simulink library "mfeval_CPI_LIB"  (R2026a)
settings: Solver=VariableStepAuto
undefined symbols (not defined in the file or in its folder): parameterStruct, userDynamics, userUseMode
Description:
  | Copyright 2020-2024 The MathWorks, Inc.
settings Model: Creator=MFURLANT  LastModifiedBy=andrei

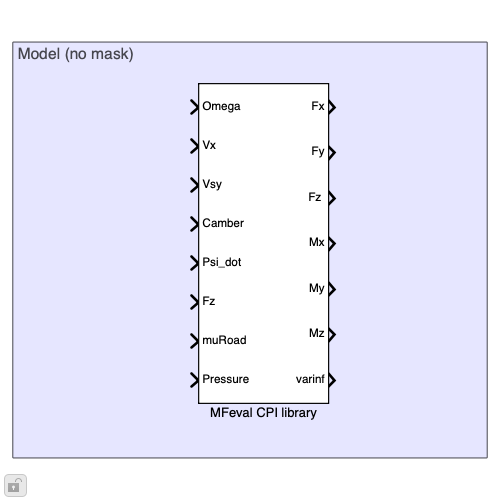
[thumbnail: Simulink's stored preview of the top-level diagram]
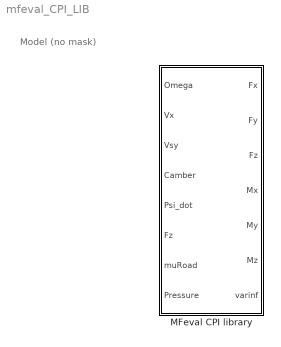
== system mfeval_CPI_LIB ==
  note: Model (no mask)
  MFeval CPI library : Subsystem

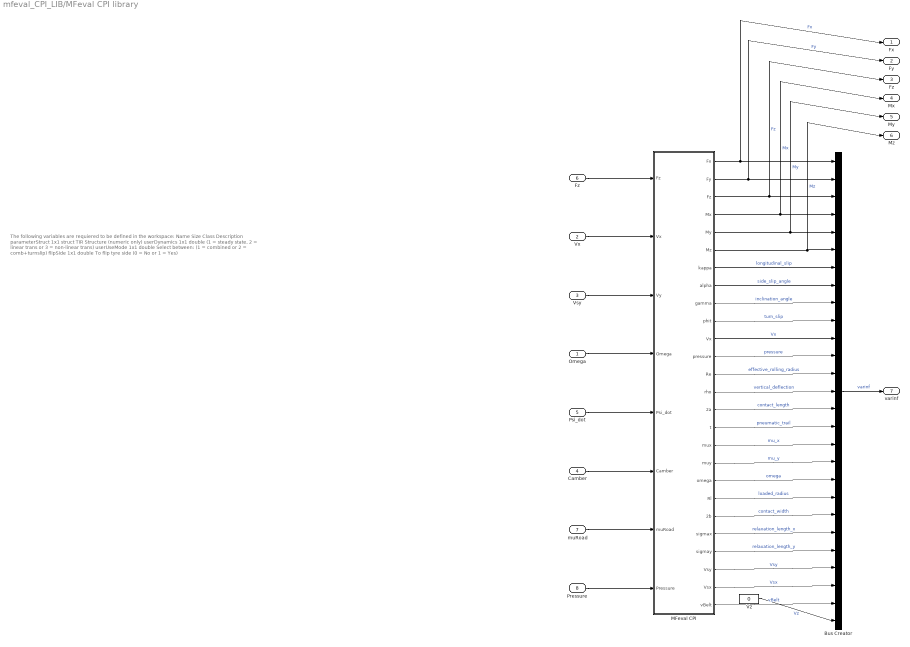
== system mfeval_CPI_LIB/MFeval CPI library ==
  note: The following variables are requiered to be defined in the workspace:
      |
      | Name
      | Size
      | Class
      | Description
      |
      | parameterStruct
      | 1x1
      | struct
      | TIR Structure (numeric only)
      |
      | userDynamics
      | 1x1
      | double
      | (1 = steady state, 2 = linear trans or 3 = non-linear trans)
      |
      | userUseMode
      | 1x1
      | double
      | Select between: (1 = combined or 2 = comb+turnslip)
      |
      | flipSide
      | 1x1
      | double
      | To flip tyre side (0 = No or 1 = Yes)
  Omega : Inport
  Vx : Inport  Port=2
  Vsy : Inport  Port=3
  Camber : Inport  Port=4
  Psi_dot : Inport  Port=5
  Fz : Inport  Port=6
  muRoad : Inport  Port=7
  Pressure : Inport  Port=8
  Bus Creator : BusCreator  Inputs=27
  MFeval CPI : Subsystem
  Vz : Constant  Value=0
  Fx : Outport  VectorParamsAs1DForOutWhenUnconnected=off
  Fy : Outport  Port=2  VectorParamsAs1DForOutWhenUnconnected=off
  "Fz " : Outport  Port=3  VectorParamsAs1DForOutWhenUnconnected=off
  Mx : Outport  Port=4  VectorParamsAs1DForOutWhenUnconnected=off
  My : Outport  Port=5  VectorParamsAs1DForOutWhenUnconnected=off
  Mz : Outport  Port=6  VectorParamsAs1DForOutWhenUnconnected=off
  varinf : Outport  Port=7  VectorParamsAs1DForOutWhenUnconnected=off
  wires:
  Vx/1 -> MFeval CPI/2(Vx)
  MFeval CPI/25(Vsx) -> Bus Creator/25  "Vsx"
  MFeval CPI/13(Re) -> Bus Creator/13  "effective_rolling_radius"
  MFeval CPI/3("Fz ") -> "Fz "/1, Bus Creator/3  "Fz"
  MFeval CPI/22(sigmax) -> Bus Creator/22  "relaxation_length_x"
  MFeval CPI/16(t) -> Bus Creator/16  "pneumatic_trail"
  MFeval CPI/4(Mx) -> Mx/1, Bus Creator/4  "Mx"
  MFeval CPI/6(Mz) -> Mz/1, Bus Creator/6  "Mz"
  MFeval CPI/17(mux) -> Bus Creator/17  "mu_x"
  Vz/1 -> Bus Creator/27  "Vz"
  MFeval CPI/21(2b) -> Bus Creator/21  "contact_width"
  MFeval CPI/1(Fx) -> Fx/1, Bus Creator/1  "Fx"
  MFeval CPI/18(muy) -> Bus Creator/18  "mu_y"
  MFeval CPI/23(sigmay) -> Bus Creator/23  "relaxation_length_y"
  MFeval CPI/8(alpha) -> Bus Creator/8  "side_slip_angle"
  MFeval CPI/7(kappa) -> Bus Creator/7  "longitudinal_slip"
  MFeval CPI/20(Rl) -> Bus Creator/20  "loaded_radius"
  MFeval CPI/15(2a) -> Bus Creator/15  "contact_length"
  MFeval CPI/19(omega) -> Bus Creator/19  "omega"
  MFeval CPI/11("Vx ") -> Bus Creator/11  "Vx"
  MFeval CPI/14(rho) -> Bus Creator/14  "vertical_deflection"
  Fz/1 -> MFeval CPI/1(Fz)
  Bus Creator/1 -> varinf/1  "varinf"
  Camber/1 -> MFeval CPI/6(Camber)
  MFeval CPI/26(vBelt) -> Bus Creator/26  "vBelt"
  MFeval CPI/9(gamma) -> Bus Creator/9  "inclination_angle"
  Omega/1 -> MFeval CPI/4(Omega)
  MFeval CPI/10(phit) -> Bus Creator/10  "turn_slip"
  MFeval CPI/24(Vsy) -> Bus Creator/24  "Vsy"
  MFeval CPI/2(Fy) -> Fy/1, Bus Creator/2  "Fy"
  Psi_dot/1 -> MFeval CPI/5(Psi_dot)
  MFeval CPI/5(My) -> My/1, Bus Creator/5  "My"
  MFeval CPI/12(pressure) -> Bus Creator/12  "pressure"
  Vsy/1 -> MFeval CPI/3(Vy)
  muRoad/1 -> MFeval CPI/7(muRoad)
  Pressure/1 -> MFeval CPI/8(Pressure)

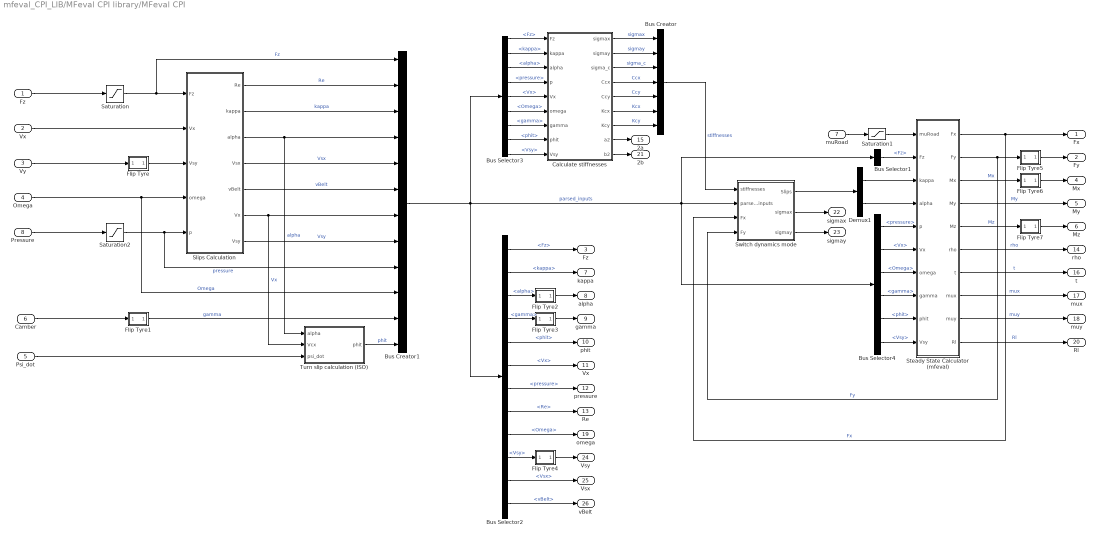
== system mfeval_CPI_LIB/MFeval CPI library/MFeval CPI ==
  Fz : Inport
  Vx : Inport  Port=2
  Vy : Inport  Port=3
  Omega : Inport  Port=4
  Psi_dot : Inport  Port=5
  Camber : Inport  Port=6
  muRoad : Inport  Port=7
  Pressure : Inport  Port=8
  Bus Creator : BusCreator  Inputs=7
  Bus Creator1 : BusCreator  Inputs=12
  Bus Selector1 : BusSelector  OutputSignals=Fz
  Bus Selector2 : BusSelector  OutputSignals=Fz,kappa,alpha,gamma,phit,Vx,pressure,Re,Omega,Vsy,Vsx,vBelt
  Bus Selector3 : BusSelector  OutputSignals=Fz,kappa,alpha,pressure,Vx,Omega,gamma,phit,Vsy
  Bus Selector4 : BusSelector  OutputSignals=pressure,Vx,Omega,gamma,phit,Vsy
  Calculate stiffnesses : MATLAB Function  TreatAsAtomicUnit=on
  Demux1 : Demux  Outputs=2
  Flip Tyre : MATLAB Function  TreatAsAtomicUnit=on
  Flip Tyre1 : MATLAB Function  TreatAsAtomicUnit=on
  Flip Tyre2 : MATLAB Function  TreatAsAtomicUnit=on
  Flip Tyre3 : MATLAB Function  TreatAsAtomicUnit=on
  Flip Tyre4 : MATLAB Function  TreatAsAtomicUnit=on
  Flip Tyre5 : MATLAB Function  TreatAsAtomicUnit=on
  Flip Tyre6 : MATLAB Function  TreatAsAtomicUnit=on
  Flip Tyre7 : MATLAB Function  TreatAsAtomicUnit=on
  Saturation : Saturate  UpperLimit=parameterStruct.FZMAX*2  LowerLimit=1e-3  ZeroCross=off
  Saturation1 : Saturate  UpperLimit=Inf  LowerLimit=0  ZeroCross=off
  Saturation2 : Saturate  UpperLimit=parameterStruct.PRESMAX  LowerLimit=parameterStruct.PRESMIN  ZeroCross=off
  Slips Calculation : MATLAB Function  TreatAsAtomicUnit=on
  Steady State Calculator (mfeval) : MATLAB Function  TreatAsAtomicUnit=on
  Switch dynamics mode : Subsystem
  Turn slip calculation (ISO) : MATLAB Function  TreatAsAtomicUnit=on
  Fx : Outport  VectorParamsAs1DForOutWhenUnconnected=off
  Fy : Outport  Port=2  VectorParamsAs1DForOutWhenUnconnected=off
  "Fz " : Outport  Port=3  VectorParamsAs1DForOutWhenUnconnected=off
  Mx : Outport  Port=4  VectorParamsAs1DForOutWhenUnconnected=off
  My : Outport  Port=5  VectorParamsAs1DForOutWhenUnconnected=off
  Mz : Outport  Port=6  VectorParamsAs1DForOutWhenUnconnected=off
  kappa : Outport  Port=7  VectorParamsAs1DForOutWhenUnconnected=off
  alpha : Outport  Port=8  VectorParamsAs1DForOutWhenUnconnected=off
  gamma : Outport  Port=9  VectorParamsAs1DForOutWhenUnconnected=off
  phit : Outport  Port=10  VectorParamsAs1DForOutWhenUnconnected=off
  "Vx " : Outport  Port=11  VectorParamsAs1DForOutWhenUnconnected=off
  pressure : Outport  Port=12  VectorParamsAs1DForOutWhenUnconnected=off
  Re : Outport  Port=13  VectorParamsAs1DForOutWhenUnconnected=off
  rho : Outport  Port=14  VectorParamsAs1DForOutWhenUnconnected=off
  2a : Outport  Port=15  VectorParamsAs1DForOutWhenUnconnected=off
  t : Outport  Port=16  VectorParamsAs1DForOutWhenUnconnected=off
  mux : Outport  Port=17  VectorParamsAs1DForOutWhenUnconnected=off
  muy : Outport  Port=18  VectorParamsAs1DForOutWhenUnconnected=off
  omega : Outport  Port=19  VectorParamsAs1DForOutWhenUnconnected=off
  Rl : Outport  Port=20  VectorParamsAs1DForOutWhenUnconnected=off
  2b : Outport  Port=21  VectorParamsAs1DForOutWhenUnconnected=off
  sigmax : Outport  Port=22  VectorParamsAs1DForOutWhenUnconnected=off
  sigmay : Outport  Port=23  VectorParamsAs1DForOutWhenUnconnected=off
  Vsy : Outport  Port=24  VectorParamsAs1DForOutWhenUnconnected=off
  Vsx : Outport  Port=25  VectorParamsAs1DForOutWhenUnconnected=off
  vBelt : Outport  Port=26  VectorParamsAs1DForOutWhenUnconnected=off
  wires:
  Pressure/1 -> Saturation2/1
  Camber/1 -> Flip Tyre1/1(in)
  Turn slip calculation (ISO)/1(phit) -> Bus Creator1/12  "phit"
  Vx/1 -> Slips Calculation/2("Vx ")
  Steady State Calculator (mfeval)/9(muy) -> muy/1  "muy"
  Steady State Calculator (mfeval)/5(Mz) -> Flip Tyre7/1(in)  "Mz"
  Vy/1 -> Flip Tyre/1(in)
  Steady State Calculator (mfeval)/3(Mx) -> Flip Tyre6/1(in)  "Mx"
  Slips Calculation/2(kappa) -> Bus Creator1/3  "kappa"
  Steady State Calculator (mfeval)/7(t) -> t/1  "t"
  Steady State Calculator (mfeval)/4(My) -> My/1  "My"
  Steady State Calculator (mfeval)/8(mux) -> mux/1  "mux"
  Steady State Calculator (mfeval)/6(rho) -> rho/1  "rho"
  Fz/1 -> Saturation/1
  Omega/1 -> Bus Creator1/10, Slips Calculation/4(omega)  "Omega"
  Psi_dot/1 -> Turn slip calculation (ISO)/3(psi_dot)
  Slips Calculation/4(Vsx) -> Bus Creator1/5  "Vsx"
  Bus Selector3/1 -> Calculate stiffnesses/1(Fz)  "<Fz>"
  Bus Selector3/2 -> Calculate stiffnesses/2(kappa)  "<kappa>"
  Bus Selector3/3 -> Calculate stiffnesses/3(alpha)  "<alpha>"
  Bus Selector3/4 -> Calculate stiffnesses/4(p)  "<pressure>"
  Bus Selector3/5 -> Calculate stiffnesses/5(Vx)  "<Vx>"
  Bus Selector3/6 -> Calculate stiffnesses/6(omega)  "<Omega>"
  Bus Selector3/7 -> Calculate stiffnesses/7(gamma)  "<gamma>"
  Bus Selector3/8 -> Calculate stiffnesses/8(phit)  "<phit>"
  Calculate stiffnesses/1(sigmax) -> Bus Creator/1  "sigmax"
  Calculate stiffnesses/2(sigmay) -> Bus Creator/2  "sigmay"
  Calculate stiffnesses/3(sigma_c) -> Bus Creator/3  "sigma_c"
  Calculate stiffnesses/4(Ccx) -> Bus Creator/4  "Ccx"
  Calculate stiffnesses/5(Ccy) -> Bus Creator/5  "Ccy"
  Calculate stiffnesses/6(Kcx) -> Bus Creator/6  "Kcx"
  Calculate stiffnesses/7(Kcy) -> Bus Creator/7  "Kcy"
  Bus Creator1/1 -> Bus Selector3/1, Bus Selector1/1, Switch dynamics mode/2(parsed_inputs), Bus Selector4/1, Bus Selector2/1  "parsed_inputs"
  Demux1/2 -> Steady State Calculator (mfeval)/4(alpha)
  Slips Calculation/3(alpha) -> Turn slip calculation (ISO)/1(alpha), Bus Creator1/4  "alpha"
  Flip Tyre2/1(out) -> alpha/1
  Flip Tyre1/1(out) -> Bus Creator1/11  "gamma"
  Flip Tyre3/1(out) -> gamma/1
  Flip Tyre6/1(out) -> Mx/1
  Flip Tyre7/1(out) -> Mz/1
  Flip Tyre5/1(out) -> Fy/1
  Flip Tyre/1(out) -> Slips Calculation/3("Vsy ")
  Flip Tyre4/1(out) -> Vsy/1
  Steady State Calculator (mfeval)/2(Fy) -> Switch dynamics mode/4(Fy), Flip Tyre5/1(in)  "Fy"
  Steady State Calculator (mfeval)/1(Fx) -> Switch dynamics mode/3(Fx), Fx/1  "Fx"
  Switch dynamics mode/1(Slips) -> Demux1/1
  Slips Calculation/6(Vx) -> Turn slip calculation (ISO)/2(Vcx), Bus Creator1/7  "Vx"
  Slips Calculation/7(Vsy) -> Bus Creator1/8  "Vsy"
  Calculate stiffnesses/8(a2) -> 2a/1
  Slips Calculation/1(Re) -> Bus Creator1/2  "Re"
  Slips Calculation/5(vBelt) -> Bus Creator1/6  "vBelt"
  Bus Selector2/1 -> "Fz "/1  "<Fz>"
  Bus Selector2/12 -> vBelt/1  "<vBelt>"
  Bus Selector2/2 -> kappa/1  "<kappa>"
  Bus Selector2/3 -> Flip Tyre2/1(in)  "<alpha>"
  Bus Selector2/4 -> Flip Tyre3/1(in)  "<gamma>"
  Bus Selector2/5 -> phit/1  "<phit>"
  Bus Selector2/6 -> "Vx "/1  "<Vx>"
  Bus Selector2/7 -> pressure/1  "<pressure>"
  Bus Selector2/8 -> Re/1  "<Re>"
  Bus Selector2/9 -> omega/1  "<Omega>"
  Bus Selector2/10 -> Flip Tyre4/1(in)  "<Vsy>"
  Bus Selector2/11 -> Vsx/1  "<Vsx>"
  Steady State Calculator (mfeval)/10(Rl) -> Rl/1  "Rl"
  Calculate stiffnesses/9(b2) -> 2b/1
  Bus Selector3/9 -> Calculate stiffnesses/9(Vsy)  "<Vsy>"
  Demux1/1 -> Steady State Calculator (mfeval)/3(kappa)
  Saturation/1 -> Bus Creator1/1, Slips Calculation/1(Fz)  "Fz"
  Bus Creator/1 -> Switch dynamics mode/1(stiffnesses)  "stiffnesses"
  Switch dynamics mode/2(sigmax) -> sigmax/1
  Switch dynamics mode/3(sigmay) -> sigmay/1
  Bus Selector1/1 -> Steady State Calculator (mfeval)/2(Fz)  "<Fz>"
  Bus Selector4/1 -> Steady State Calculator (mfeval)/5(p)  "<pressure>"
  Bus Selector4/2 -> Steady State Calculator (mfeval)/6(Vx)  "<Vx>"
  Bus Selector4/3 -> Steady State Calculator (mfeval)/7(omega)  "<Omega>"
  Bus Selector4/4 -> Steady State Calculator (mfeval)/8(gamma)  "<gamma>"
  Bus Selector4/5 -> Steady State Calculator (mfeval)/9(phit)  "<phit>"
  Bus Selector4/6 -> Steady State Calculator (mfeval)/10(Vsy)  "<Vsy>"
  muRoad/1 -> Saturation1/1
  Saturation1/1 -> Steady State Calculator (mfeval)/1(muRoad)
  Saturation2/1 -> Bus Creator1/9, Slips Calculation/5(p)  "pressure"

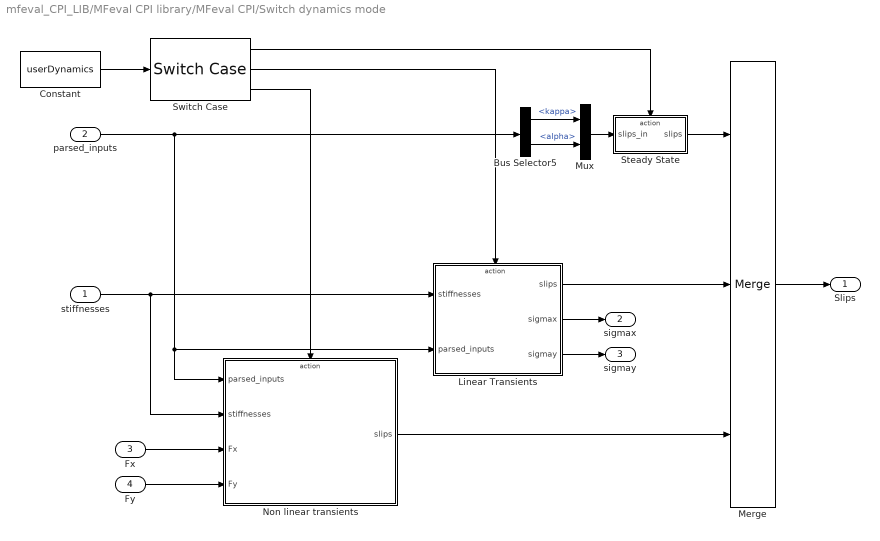
== system mfeval_CPI_LIB/MFeval CPI library/MFeval CPI/Switch dynamics mode ==
  stiffnesses : Inport
  parsed_inputs : Inport  Port=2
  Fx : Inport  Port=3
  Fy : Inport  Port=4
  Bus Selector5 : BusSelector  OutputSignals=kappa,alpha
  Constant : Constant  Value=userDynamics
  Linear Transients : Subsystem  TreatAsAtomicUnit=on
  Merge : Merge  Inputs=3
  Mux : Mux  Inputs=2
  Non linear transients : Subsystem  TreatAsAtomicUnit=on
  Steady State : Subsystem  TreatAsAtomicUnit=on
  Switch Case : SwitchCase  CaseConditions={1, 2}
  Slips : Outport  VectorParamsAs1DForOutWhenUnconnected=off
  sigmax : Outport  Port=2  VectorParamsAs1DForOutWhenUnconnected=off
  sigmay : Outport  Port=3  VectorParamsAs1DForOutWhenUnconnected=off
  wires:
  Constant/1 -> Switch Case/1
  Switch Case/1 -> Steady State/Action
  Switch Case/2 -> Linear Transients/Action
  Linear Transients/1(slips) -> Merge/2
  Switch Case/3 -> Non linear transients/Action
  Non linear transients/1(slips) -> Merge/3
  Steady State/1(slips) -> Merge/1
  Merge/1 -> Slips/1
  parsed_inputs/1 -> Bus Selector5/1, Non linear transients/1(parsed_inputs), Linear Transients/2(parsed_inputs)
  Fx/1 -> Non linear transients/3(Fx)
  Fy/1 -> Non linear transients/4(Fy)
  stiffnesses/1 -> Non linear transients/2(stiffnesses), Linear Transients/1(stiffnesses)
  Linear Transients/2(sigmax) -> sigmax/1
  Linear Transients/3(sigmay) -> sigmay/1
  Bus Selector5/2 -> Mux/2  "<alpha>"
  Bus Selector5/1 -> Mux/1  "<kappa>"
  Mux/1 -> Steady State/1(slips_in)

== system mfeval_CPI_LIB/MFeval CPI library/MFeval CPI/Switch dynamics mode/Linear Transients ==
  stiffnesses : Inport
  parsed_inputs : Inport  Port=2
  Action Port : ActionPort  ActionPortLabel=case: { }
  Bus Selector : BusSelector  OutputSignals=sigmax,sigmay
  Bus Selector5 : BusSelector  OutputSignals=Vsx,Vsy,Vx
  Calculate Slips : Subsystem  TreatAsAtomicUnit=on
  Mux1 : Mux  Inputs=2
  slips : Outport  VectorParamsAs1DForOutWhenUnconnected=off
  sigmax : Outport  Port=2  VectorParamsAs1DForOutWhenUnconnected=off
  sigmay : Outport  Port=3  VectorParamsAs1DForOutWhenUnconnected=off
  wires:
  Calculate Slips/2(alpha) -> Mux1/2
  Mux1/1 -> slips/1  "Linear transients"
  Bus Selector/2 -> sigmay/1, Calculate Slips/2(sigmay)  "<sigmay>"
  Bus Selector5/3 -> Calculate Slips/5(Vx)  "<Vx>"
  Calculate Slips/1(kappa) -> Mux1/1
  Bus Selector5/2 -> Calculate Slips/4(Vsy)  "<Vsy>"
  Bus Selector5/1 -> Calculate Slips/3(Vsx)  "<Vsx>"
  Bus Selector/1 -> sigmax/1, Calculate Slips/1(sigmax)  "<sigmax>"
  stiffnesses/1 -> Bus Selector/1  "stiffnesses"
  parsed_inputs/1 -> Bus Selector5/1

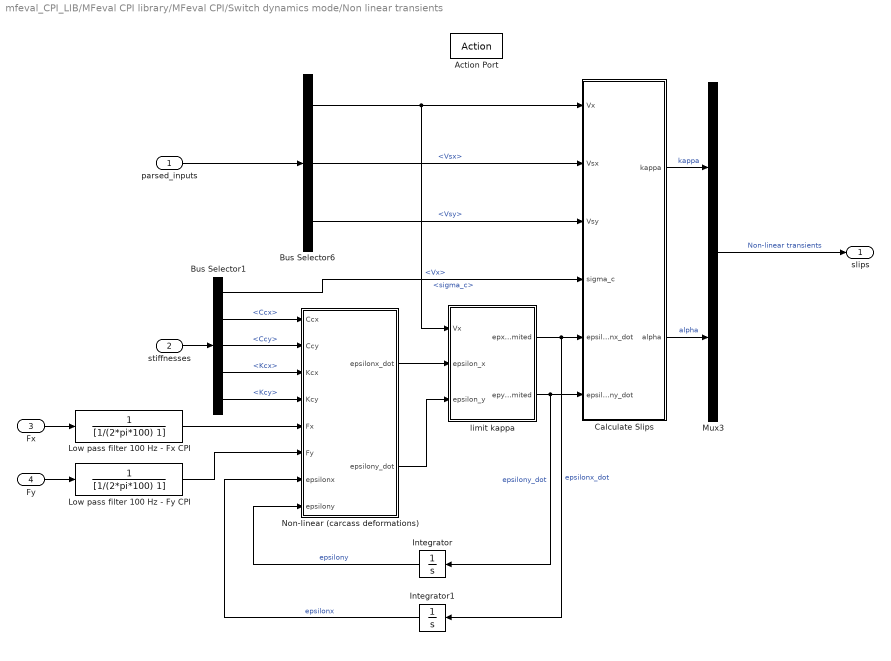
== system mfeval_CPI_LIB/MFeval CPI library/MFeval CPI/Switch dynamics mode/Non linear transients ==
  parsed_inputs : Inport
  stiffnesses : Inport  Port=2
  Fx : Inport  Port=3
  Fy : Inport  Port=4
  Action Port : ActionPort  ActionPortLabel=default: { }
  Bus Selector1 : BusSelector  OutputSignals=sigma_c,Ccx,Ccy,Kcx,Kcy
  Bus Selector6 : BusSelector  OutputSignals=Vx,Vsx,Vsy
  Calculate Slips : Subsystem  TreatAsAtomicUnit=on
  Integrator : Integrator
  Integrator1 : Integrator
  Low pass filter 100 Hz - Fx CPI : TransferFcn  Denominator=[1/(2*pi*100) 1]
  Low pass filter 100 Hz - Fy CPI : TransferFcn  Denominator=[1/(2*pi*100) 1]
  Mux3 : Mux  Inputs=2
  Non-linear (carcass deformations) : Subsystem
  limit kappa : Subsystem
  slips : Outport  VectorParamsAs1DForOutWhenUnconnected=off
  wires:
  Calculate Slips/1(kappa) -> Mux3/1  "kappa"
  Mux3/1 -> slips/1  "Non-linear transients"
  Non-linear (carcass deformations)/1(epsilonx_dot) -> limit kappa/2(epsilon_x)
  Bus Selector1/5 -> Non-linear (carcass deformations)/4(Kcy)  "<Kcy>"
  Bus Selector6/2 -> Calculate Slips/2(Vsx)  "<Vsx>"
  Integrator/1 -> Non-linear (carcass deformations)/8(epsilony)  "epsilony"
  Bus Selector1/4 -> Non-linear (carcass deformations)/3(Kcx)  "<Kcx>"
  Calculate Slips/2(alpha) -> Mux3/2  "alpha"
  Non-linear (carcass deformations)/2(epsilony_dot) -> limit kappa/3(epsilon_y)
  Bus Selector6/1 -> limit kappa/1(Vx), Calculate Slips/1(Vx)  "<Vx>"
  limit kappa/2(epy_limited) -> Integrator/1, Calculate Slips/6(epsilony_dot)  "epsilony_dot"
  Bus Selector6/3 -> Calculate Slips/3(Vsy)  "<Vsy>"
  Bus Selector1/2 -> Non-linear (carcass deformations)/1(Ccx)  "<Ccx>"
  Integrator1/1 -> Non-linear (carcass deformations)/7(epsilonx)  "epsilonx"
  Bus Selector1/3 -> Non-linear (carcass deformations)/2(Ccy)  "<Ccy>"
  Bus Selector1/1 -> Calculate Slips/4(sigma_c)  "<sigma_c>"
  limit kappa/1(epx_limited) -> Integrator1/1, Calculate Slips/5(epsilonx_dot)  "epsilonx_dot"
  parsed_inputs/1 -> Bus Selector6/1
  stiffnesses/1 -> Bus Selector1/1
  Fx/1 -> Low pass filter 100 Hz - Fx CPI/1
  Fy/1 -> Low pass filter 100 Hz - Fy CPI/1
  Low pass filter 100 Hz - Fy CPI/1 -> Non-linear (carcass deformations)/6(Fy)
  Low pass filter 100 Hz - Fx CPI/1 -> Non-linear (carcass deformations)/5(Fx)

== system mfeval_CPI_LIB/MFeval CPI library/MFeval CPI/Switch dynamics mode/Steady State ==
  slips_in : Inport
  Action Port : ActionPort  ActionPortLabel=case: { }
  slips : Outport  VectorParamsAs1DForOutWhenUnconnected=off
  wires:
  slips_in/1 -> slips/1

== system mfeval_CPI_LIB/MFeval CPI library/MFeval CPI/Switch dynamics mode/Linear Transients/Calculate Slips ==
  sigmax : Inport
  sigmay : Inport  Port=2
  Vsx : Inport  Port=3
  Vsy : Inport  Port=4
  Vx : Inport  Port=5
  Integrator : Integrator
  Integrator1 : Integrator
  calculate alpha_dot : Subsystem
  calculate kappa_dot : Subsystem
  kappa : Outport  VectorParamsAs1DForOutWhenUnconnected=off
  alpha : Outport  Port=2  VectorParamsAs1DForOutWhenUnconnected=off
  wires:
  Vx/1 -> calculate kappa_dot/1(Vx), calculate alpha_dot/1(Vx)
  Integrator1/1 -> kappa/1, calculate kappa_dot/4(kappa)  "kappa"
  Integrator/1 -> alpha/1, calculate alpha_dot/4(alpha)  "alpha"
  calculate kappa_dot/1(kappa_dot) -> Integrator1/1  "kappa_dot"
  calculate alpha_dot/1(alpha_dot) -> Integrator/1  "alpha_dot"
  sigmax/1 -> calculate kappa_dot/3(sigmax)
  Vsy/1 -> calculate alpha_dot/2(Vsy)
  sigmay/1 -> calculate alpha_dot/3(sigmay)
  Vsx/1 -> calculate kappa_dot/2(Vsx)

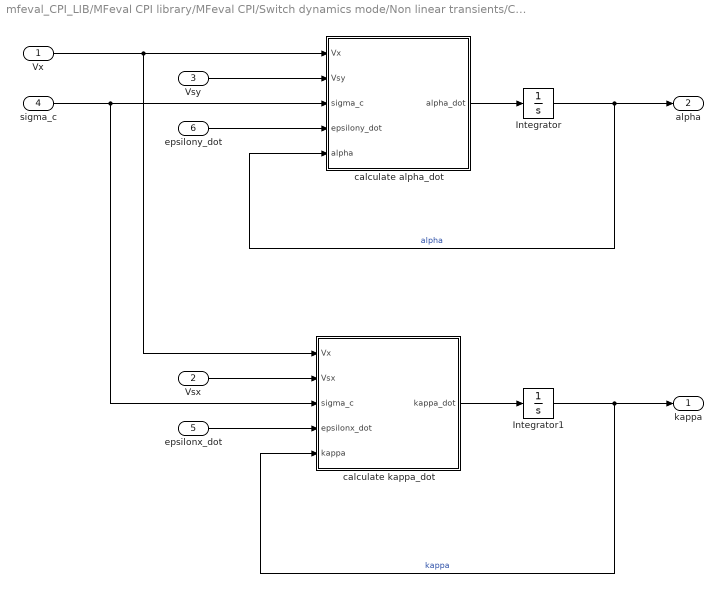
== system mfeval_CPI_LIB/MFeval CPI library/MFeval CPI/Switch dynamics mode/Non linear transients/Calculate Slips ==
  Vx : Inport
  Vsx : Inport  Port=2
  Vsy : Inport  Port=3
  sigma_c : Inport  Port=4
  epsilonx_dot : Inport  Port=5
  epsilony_dot : Inport  Port=6
  Integrator : Integrator
  Integrator1 : Integrator
  calculate alpha_dot : Subsystem
  calculate kappa_dot : Subsystem
  kappa : Outport  VectorParamsAs1DForOutWhenUnconnected=off
  alpha : Outport  Port=2  VectorParamsAs1DForOutWhenUnconnected=off
  wires:
  Integrator1/1 -> calculate kappa_dot/5(kappa), kappa/1  "kappa"
  Integrator/1 -> calculate alpha_dot/5(alpha), alpha/1  "alpha"
  epsilony_dot/1 -> calculate alpha_dot/4(epsilony_dot)
  calculate alpha_dot/1(alpha_dot) -> Integrator/1
  calculate kappa_dot/1(kappa_dot) -> Integrator1/1
  sigma_c/1 -> calculate kappa_dot/3(sigma_c), calculate alpha_dot/3(sigma_c)
  Vsy/1 -> calculate alpha_dot/2(Vsy)
  Vsx/1 -> calculate kappa_dot/2(Vsx)
  epsilonx_dot/1 -> calculate kappa_dot/4(epsilonx_dot)
  Vx/1 -> calculate kappa_dot/1(Vx), calculate alpha_dot/1(Vx)

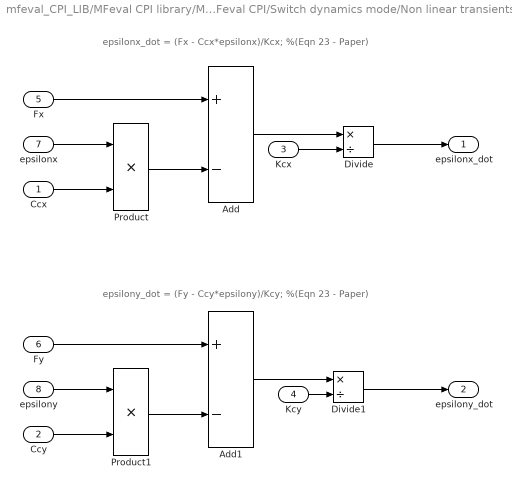
== system mfeval_CPI_LIB/MFeval CPI library/MFeval CPI/Switch dynamics mode/Non linear transients/Non-linear (carcass deformations) ==
  note: epsilony_dot = (Fy - Ccy*epsilony)/Kcy; %(Eqn 23 - Paper)
  note: epsilonx_dot = (Fx - Ccx*epsilonx)/Kcx; %(Eqn 23 - Paper)
  Ccx : Inport
  Ccy : Inport  Port=2
  Kcx : Inport  Port=3
  Kcy : Inport  Port=4
  Fx : Inport  Port=5
  Fy : Inport  Port=6
  epsilonx : Inport  Port=7
  epsilony : Inport  Port=8
  Add : Sum  Inputs=+-
  Add1 : Sum  Inputs=+-
  Divide : Product  Inputs=*/
  Divide1 : Product  Inputs=*/
  Product : Product
  Product1 : Product
  epsilonx_dot : Outport  VectorParamsAs1DForOutWhenUnconnected=off
  epsilony_dot : Outport  Port=2  VectorParamsAs1DForOutWhenUnconnected=off
  wires:
  Fx/1 -> Add/1
  epsilonx/1 -> Product/1
  Ccx/1 -> Product/2
  Product/1 -> Add/2
  Add/1 -> Divide/1
  Kcx/1 -> Divide/2
  Divide/1 -> epsilonx_dot/1
  Ccy/1 -> Product1/2
  epsilony/1 -> Product1/1
  Product1/1 -> Add1/2
  Fy/1 -> Add1/1
  Add1/1 -> Divide1/1
  Kcy/1 -> Divide1/2
  Divide1/1 -> epsilony_dot/1

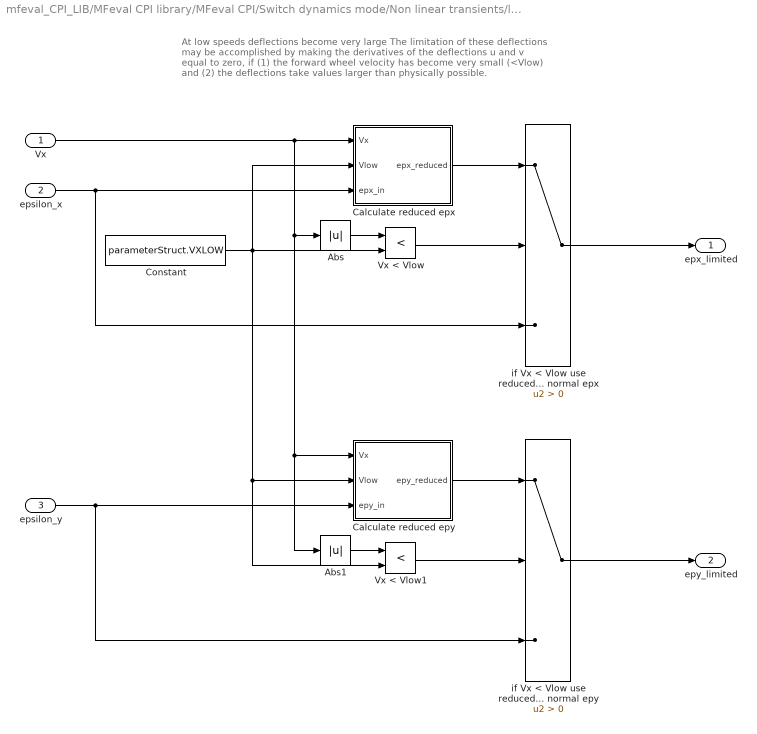
== system mfeval_CPI_LIB/MFeval CPI library/MFeval CPI/Switch dynamics mode/Non linear transients/limit kappa ==
  note: At low speeds deflections become very large
      | The limitation of these deflections may be accomplished by making the
      | derivatives of the deflections u and v equal to zero, if (1) the forward
      | wheel velocity has become very small (<Vlow) and (2) the deflections take
      | values larger than physically possible.
  Vx : Inport
  epsilon_x : Inport  Port=2
  epsilon_y : Inport  Port=3
  Abs : Abs  ZeroCross=off  SaturateOnIntegerOverflow=off
  Abs1 : Abs  ZeroCross=off  SaturateOnIntegerOverflow=off
  Calculate reduced epx : Subsystem
  Calculate reduced epy : Subsystem
  Constant : Constant  Value=parameterStruct.VXLOW
  Vx < Vlow : RelationalOperator  Operator=<  OutDataTypeStr=boolean  ZeroCross=off  RndMeth=Simplest  InputSameDT=off
  Vx < Vlow1 : RelationalOperator  Operator=<  OutDataTypeStr=boolean  ZeroCross=off  RndMeth=Simplest  InputSameDT=off
  if Vx < Vlow use reduced epx else normal epx : Switch  Criteria=u2 > Threshold  SaturateOnIntegerOverflow=off  InputSameDT=off
  if Vx < Vlow use reduced epy else normal epy : Switch  Criteria=u2 > Threshold  SaturateOnIntegerOverflow=off  InputSameDT=off
  epx_limited : Outport  VectorParamsAs1DForOutWhenUnconnected=off
  epy_limited : Outport  Port=2  VectorParamsAs1DForOutWhenUnconnected=off
  wires:
  epsilon_x/1 -> Calculate reduced epx/3(epx_in), if Vx < Vlow use reduced epx else normal epx/3
  if Vx < Vlow use reduced epx else normal epx/1 -> epx_limited/1
  Vx/1 -> Calculate reduced epx/1(Vx), Abs1/1, Calculate reduced epy/1(Vx), Abs/1
  Calculate reduced epx/1(epx_reduced) -> if Vx < Vlow use reduced epx else normal epx/1
  Vx < Vlow/1 -> if Vx < Vlow use reduced epx else normal epx/2
  Calculate reduced epy/1(epy_reduced) -> if Vx < Vlow use reduced epy else normal epy/1
  epsilon_y/1 -> Calculate reduced epy/3(epy_in), if Vx < Vlow use reduced epy else normal epy/3
  Constant/1 -> Vx < Vlow1/2, Calculate reduced epy/2(Vlow), Calculate reduced epx/2(Vlow), Vx < Vlow/2
  if Vx < Vlow use reduced epy else normal epy/1 -> epy_limited/1
  Vx < Vlow1/1 -> if Vx < Vlow use reduced epy else normal epy/2
  Abs/1 -> Vx < Vlow/1
  Abs1/1 -> Vx < Vlow1/1

== system mfeval_CPI_LIB/MFeval CPI library/MFeval CPI/Switch dynamics mode/Linear Transients/Calculate Slips/calculate alpha_dot ==
  note: alpha_dot = (-abs(Vx).*alpha + Vsy)./ max(sigmay, 0.02); % (Eqn 21 - Paper)
  Vx : Inport
  Vsy : Inport  Port=2
  sigmay : Inport  Port=3
  alpha : Inport  Port=4
  Abs : Abs  ZeroCross=off  SaturateOnIntegerOverflow=off
  Add : Sum
  Constant : Constant  Value=0.02
  Divide : Product  Inputs=*/
  Gain : Gain  Gain=-1
  MinMax : MinMax  Function=max  Inputs=2  ZeroCross=off
  Product : Product
  alpha_dot : Outport  VectorParamsAs1DForOutWhenUnconnected=off
  wires:
  Vx/1 -> Abs/1
  alpha/1 -> Product/2
  Abs/1 -> Gain/1
  Product/1 -> Add/1
  Vsy/1 -> Add/2
  Add/1 -> Divide/1
  sigmay/1 -> MinMax/2
  MinMax/1 -> Divide/2
  Constant/1 -> MinMax/1
  Divide/1 -> alpha_dot/1
  Gain/1 -> Product/1

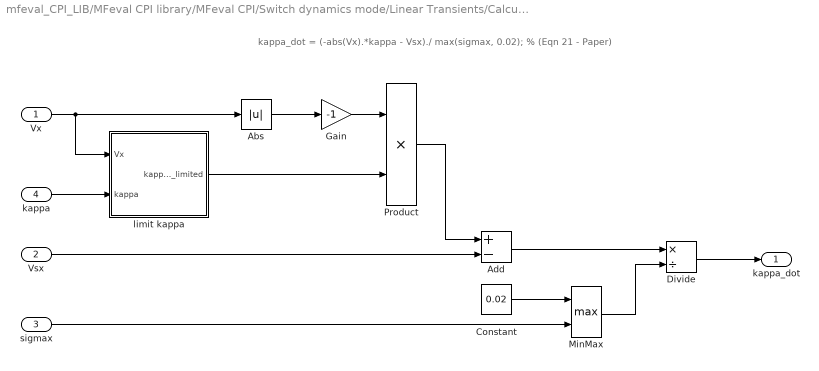
== system mfeval_CPI_LIB/MFeval CPI library/MFeval CPI/Switch dynamics mode/Linear Transients/Calculate Slips/calculate kappa_dot ==
  note: kappa_dot = (-abs(Vx).*kappa - Vsx)./ max(sigmax, 0.02); % (Eqn 21 - Paper)
  Vx : Inport
  Vsx : Inport  Port=2
  sigmax : Inport  Port=3
  kappa : Inport  Port=4
  Abs : Abs  ZeroCross=off  SaturateOnIntegerOverflow=off
  Add : Sum  Inputs=+-
  Constant : Constant  Value=0.02
  Divide : Product  Inputs=*/
  Gain : Gain  Gain=-1
  MinMax : MinMax  Function=max  Inputs=2  ZeroCross=off
  Product : Product
  limit kappa : Subsystem
  kappa_dot : Outport  VectorParamsAs1DForOutWhenUnconnected=off
  wires:
  MinMax/1 -> Divide/2
  Gain/1 -> Product/1
  Constant/1 -> MinMax/1
  Product/1 -> Add/1
  Divide/1 -> kappa_dot/1
  Vsx/1 -> Add/2
  sigmax/1 -> MinMax/2
  Add/1 -> Divide/1
  Abs/1 -> Gain/1
  kappa/1 -> limit kappa/2(kappa)
  Vx/1 -> limit kappa/1(Vx), Abs/1
  limit kappa/1(kappa_limited) -> Product/2

== system mfeval_CPI_LIB/MFeval CPI library/MFeval CPI/Switch dynamics mode/Non linear transients/Calculate Slips/calculate alpha_dot ==
  note: alpha_dot = (-abs(Vx)*alpha + Vsy + epsilony_dot)/ sigma_c; % (Eqn 21 - Paper)
  Vx : Inport
  Vsy : Inport  Port=2
  sigma_c : Inport  Port=3
  epsilony_dot : Inport  Port=4
  alpha : Inport  Port=5
  Abs : Abs  ZeroCross=off  SaturateOnIntegerOverflow=off
  Add : Sum  Inputs=+++
  Divide : Product  Inputs=*/
  Gain : Gain  Gain=-1
  Product : Product
  alpha_dot : Outport  VectorParamsAs1DForOutWhenUnconnected=off
  wires:
  Vx/1 -> Abs/1
  Gain/1 -> Product/1
  Abs/1 -> Gain/1
  alpha/1 -> Product/2
  Product/1 -> Add/1
  Vsy/1 -> Add/2
  epsilony_dot/1 -> Add/3
  Add/1 -> Divide/1
  sigma_c/1 -> Divide/2
  Divide/1 -> alpha_dot/1

== system mfeval_CPI_LIB/MFeval CPI library/MFeval CPI/Switch dynamics mode/Non linear transients/Calculate Slips/calculate kappa_dot ==
  note: kappa_dot = (-abs(Vx).*kappa - (Vsx + epsilonx_dot))./ sigma_c; % (Eqn 21 - Paper)
  Vx : Inport
  Vsx : Inport  Port=2
  sigma_c : Inport  Port=3
  epsilonx_dot : Inport  Port=4
  kappa : Inport  Port=5
  Abs : Abs  ZeroCross=off  SaturateOnIntegerOverflow=off
  Add : Sum
  Add1 : Sum  Inputs=+-
  Divide : Product  Inputs=*/
  Gain : Gain  Gain=-1
  Product : Product
  kappa_dot : Outport  VectorParamsAs1DForOutWhenUnconnected=off
  wires:
  Divide/1 -> kappa_dot/1
  sigma_c/1 -> Divide/2
  Add1/1 -> Divide/1
  epsilonx_dot/1 -> Add/2
  Vsx/1 -> Add/1
  Product/1 -> Add1/1
  kappa/1 -> Product/2
  Abs/1 -> Gain/1
  Gain/1 -> Product/1
  Vx/1 -> Abs/1
  Add/1 -> Add1/2

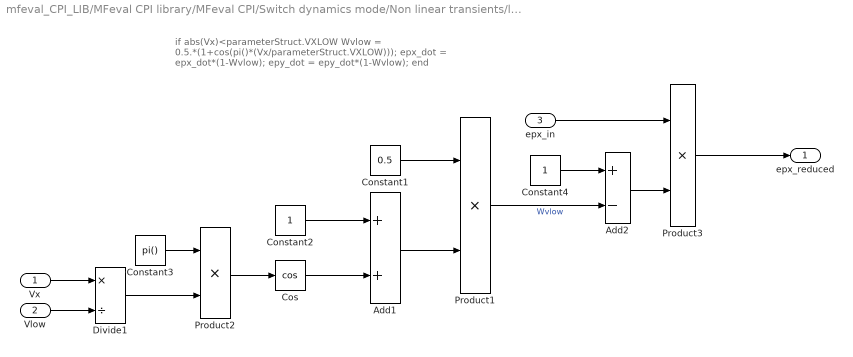
== system mfeval_CPI_LIB/MFeval CPI library/MFeval CPI/Switch dynamics mode/Non linear transients/limit kappa/Calculate reduced epx ==
  note: if abs(Vx)<parameterStruct.VXLOW
      |     Wvlow = 0.5.*(1+cos(pi()*(Vx/parameterStruct.VXLOW)));
      |     epx_dot = epx_dot*(1-Wvlow);
      |     epy_dot = epy_dot*(1-Wvlow);
      | end
  Vx : Inport
  Vlow : Inport  Port=2
  epx_in : Inport  Port=3
  Add1 : Sum
  Add2 : Sum  Inputs=+-
  Constant1 : Constant  Value=0.5
  Constant2 : Constant
  Constant3 : Constant  Value=pi()
  Constant4 : Constant
  Cos : Trigonometry  Operator=cos
  Divide1 : Product  Inputs=*/
  Product1 : Product
  Product2 : Product
  Product3 : Product
  epx_reduced : Outport  VectorParamsAs1DForOutWhenUnconnected=off
  wires:
  Product2/1 -> Cos/1
  Add2/1 -> Product3/2
  Constant3/1 -> Product2/1
  Vlow/1 -> Divide1/2
  Product3/1 -> epx_reduced/1
  Constant2/1 -> Add1/1
  Product1/1 -> Add2/2  "Wvlow"
  epx_in/1 -> Product3/1
  Cos/1 -> Add1/2
  Add1/1 -> Product1/2
  Constant4/1 -> Add2/1
  Divide1/1 -> Product2/2
  Vx/1 -> Divide1/1
  Constant1/1 -> Product1/1

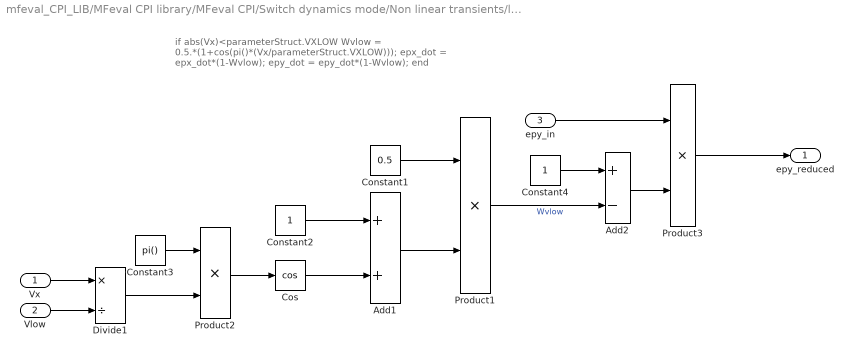
== system mfeval_CPI_LIB/MFeval CPI library/MFeval CPI/Switch dynamics mode/Non linear transients/limit kappa/Calculate reduced epy ==
  note: if abs(Vx)<parameterStruct.VXLOW
      |     Wvlow = 0.5.*(1+cos(pi()*(Vx/parameterStruct.VXLOW)));
      |     epx_dot = epx_dot*(1-Wvlow);
      |     epy_dot = epy_dot*(1-Wvlow);
      | end
  Vx : Inport
  Vlow : Inport  Port=2
  epy_in : Inport  Port=3
  Add1 : Sum
  Add2 : Sum  Inputs=+-
  Constant1 : Constant  Value=0.5
  Constant2 : Constant
  Constant3 : Constant  Value=pi()
  Constant4 : Constant
  Cos : Trigonometry  Operator=cos
  Divide1 : Product  Inputs=*/
  Product1 : Product
  Product2 : Product
  Product3 : Product
  epy_reduced : Outport  VectorParamsAs1DForOutWhenUnconnected=off
  wires:
  Product2/1 -> Cos/1
  Add2/1 -> Product3/2
  Constant3/1 -> Product2/1
  Vlow/1 -> Divide1/2
  Product3/1 -> epy_reduced/1
  Constant2/1 -> Add1/1
  Product1/1 -> Add2/2  "Wvlow"
  epy_in/1 -> Product3/1
  Cos/1 -> Add1/2
  Add1/1 -> Product1/2
  Constant4/1 -> Add2/1
  Divide1/1 -> Product2/2
  Vx/1 -> Divide1/1
  Constant1/1 -> Product1/1

== system mfeval_CPI_LIB/MFeval CPI library/MFeval CPI/Switch dynamics mode/Linear Transients/Calculate Slips/calculate kappa_dot/limit kappa ==
  note: if abs(Vx)<parameterStruct.VXLOW
      |     Wvlow = 0.5.*(1+cos(pi()*(Vx/parameterStruct.VXLOW)));
      |     kappa = kappa*(1-Wvlow);
      | end
  Vx : Inport
  kappa : Inport  Port=2
  Abs : Abs  ZeroCross=off  SaturateOnIntegerOverflow=off
  Calculate reduced kappa : Subsystem
  Constant : Constant  Value=parameterStruct.VXLOW
  Vx < Vlow : RelationalOperator  Operator=<  OutDataTypeStr=boolean  ZeroCross=off  RndMeth=Simplest  InputSameDT=off
  if Vx < Vlow use reduced kappa else normal kappa : Switch  Criteria=u2 > Threshold  SaturateOnIntegerOverflow=off  InputSameDT=off
  kappa_limited : Outport  VectorParamsAs1DForOutWhenUnconnected=off
  wires:
  Constant/1 -> Calculate reduced kappa/2(Vlow), Vx < Vlow/2
  kappa/1 -> Calculate reduced kappa/3(kappa_in), if Vx < Vlow use reduced kappa else normal kappa/3
  if Vx < Vlow use reduced kappa else normal kappa/1 -> kappa_limited/1
  Vx/1 -> Calculate reduced kappa/1(Vx), Abs/1
  Calculate reduced kappa/1(kappa_reduced) -> if Vx < Vlow use reduced kappa else normal kappa/1
  Vx < Vlow/1 -> if Vx < Vlow use reduced kappa else normal kappa/2
  Abs/1 -> Vx < Vlow/1

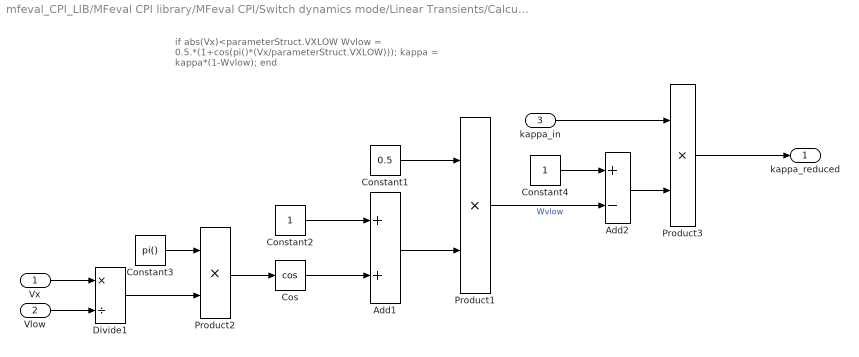
== system mfeval_CPI_LIB/MFeval CPI library/MFeval CPI/Switch dynamics mode/Linear Transients/Calculate Slips/calculate kappa_dot/limit kappa/Calculate reduced kappa ==
  note: if abs(Vx)<parameterStruct.VXLOW
      |     Wvlow = 0.5.*(1+cos(pi()*(Vx/parameterStruct.VXLOW)));
      |     kappa = kappa*(1-Wvlow);
      | end
  Vx : Inport
  Vlow : Inport  Port=2
  kappa_in : Inport  Port=3
  Add1 : Sum
  Add2 : Sum  Inputs=+-
  Constant1 : Constant  Value=0.5
  Constant2 : Constant
  Constant3 : Constant  Value=pi()
  Constant4 : Constant
  Cos : Trigonometry  Operator=cos
  Divide1 : Product  Inputs=*/
  Product1 : Product
  Product2 : Product
  Product3 : Product
  kappa_reduced : Outport  VectorParamsAs1DForOutWhenUnconnected=off
  wires:
  Product2/1 -> Cos/1
  Add2/1 -> Product3/2
  Constant3/1 -> Product2/1
  Vlow/1 -> Divide1/2
  Product3/1 -> kappa_reduced/1
  Constant2/1 -> Add1/1
  Product1/1 -> Add2/2  "Wvlow"
  kappa_in/1 -> Product3/1
  Cos/1 -> Add1/2
  Add1/1 -> Product1/2
  Constant4/1 -> Add2/1
  Divide1/1 -> Product2/2
  Vx/1 -> Divide1/1
  Constant1/1 -> Product1/1

== matlab function mfeval_CPI_LIB/MFeval CPI library/MFeval CPI/Flip Tyre5 ==
  data: in input; flipSide parameter; out output
function out = flipsSide(in, flipSide)
%#codegen

if flipSide
    out = -in;
else
    out = in;
end

== matlab function mfeval_CPI_LIB/MFeval CPI library/MFeval CPI/Flip Tyre6 ==
  data: in input; flipSide parameter; out output
function out = flipsSide(in, flipSide)
%#codegen

if flipSide
    out = -in;
else
    out = in;
end

== matlab function mfeval_CPI_LIB/MFeval CPI library/MFeval CPI/Slips Calculation ==
  data: Re output; Fz input; kappa output; Vx input; Vsy input; omega input; alpha output; p input; parameterStruct parameter; Vsx output; vBelt output; Vx output; Vsy output
function [Re, kappa, alpha, Vsx, vBelt, Vx, Vsy] = calcSlips(Fz, Vx, Vsy, omega, p,parameterStruct)
%#codegen

% Get norminal pressure
pio = parameterStruct.NOMPRES; % Reference pressure

% Normalized change in inflation pressure
dpi = (p - pio)./pio; % [Eqn (4.E2b) Page 177 - Book]

% Pack the inputs:
postProInputs.uVcx = Vx;
postProInputs.uFz = Fz;
postProInputs.omega = omega;
postProInputs.nInputs = 8;
postProInputs.ukappa = 0; % Not used but required for code generation

% Call mfeval to calculate the effective radius
solver = mfeval.Solver;
[Re, ~, ~] = solver.calculateRe(parameterStruct, postProInputs, dpi);

% Longitudinal slip velocity
Vsx = Vx - Re.*omega; % [Eqn (2.3) Page 64 - Book]

% IPG CarMaker quantity
vBelt = Re.*omega;

% Check if is low speed
isLowSpeed = abs(Vx) < parameterStruct.VXLOW;

if isLowSpeed
    % Avoid sign(0) = 0
    signVx = sign(Vx);
    signVx(signVx == 0) = 1;
   
    % Low speed Slip Ratio Calculation
    kappa = -(Vsx) * signVx;
else
    % Slip Ratio Calculation
    kappa = -(Vsx./Vx); % [Eqn (2.4) Page 64 - Book]
end

if isnan(kappa)
    kappa = 0;
end

% Slip Angle
alpha = atan(Vsy./abs(Vx)); % [Eqn (2.9) Page 67 - Book]

if isnan(alpha)
    alpha = 0;
end

% Important Note:
% Due to the ISO sign convention, equation 2.9 does not need a
% negative sign. The pacejka book is written in adapted SAE.

== matlab function mfeval_CPI_LIB/MFeval CPI library/MFeval CPI/Turn slip calculation (ISO) ==
  data: alpha input; Vcx input; psi_dot input; phit output; parameterStruct parameter
function phit  = calcTurnSlip(alpha, Vcx, psi_dot, parameterStruct)
%#codegen

% Low speed check
VXLOW = parameterStruct.VXLOW;
isLowSpeed = abs(Vcx) < VXLOW;

% if the speed is zero, avoid zero division
Vcx(Vcx==0) = 1e-6;

% IMPORTANT NOTE: Empirically discovered that TNO Simulink do not use the
% protected speed Vc_prime.

% Calculate phit
phit = -psi_dot./Vcx; % [Eqn (4.75) Page 183 - Book]

% Correction of phit with alpha (Empirically discovered)
phit= phit.*cos(alpha); 

% If the speed is negative, the turn slip is also negative
phit(Vcx<0) = -phit(Vcx<0);

% If Vcx is close to zero, use linear degression
phit(isLowSpeed) = phit(isLowSpeed).*(abs(Vcx(isLowSpeed))./VXLOW);

== matlab function mfeval_CPI_LIB/MFeval CPI library/MFeval CPI/Calculate stiffnesses ==
  data: sigmax output; sigmay output; Fz input; kappa input; alpha input; p input; Vx input; omega input; gamma input; phit input; Vsy input; userUseMode parameter; sigma_c output; parameterStruct parameter; Ccx output; Ccy output; Kcx output; Kcy output; a2 output; b2 output; userDynamics parameter
function [sigmax, sigmay, sigma_c, Ccx, Ccy, Kcx, Kcy, a2, b2] = parseInputs(Fz, kappa, alpha, p, Vx, omega, gamma, phit, Vsy, userUseMode, parameterStruct, userDynamics)
%#codegen

% Get the right useMode number
if userUseMode>1
    useMode = 212;
else
    useMode = 211;
end

% Limit Fz to avoid Infs with variable solvers
if Fz<=1e-3
    Fz = 1e-3;
elseif Fz>parameterStruct.FZMAX*2
    Fz = parameterStruct.FZMAX*2;
end

% Create the inputs
inputs = [Fz, kappa, alpha, gamma, phit, Vx, p, omega, Vsy];

% Parse inputs
solver = mfeval.Solver;
[postProInputs, internalParams, useModes] = solver.parseInputs(parameterStruct, inputs, useMode, userDynamics);

% Calculate star and prime variables
[starVar, primeVar, incrVar, ~] = solver.calculateBasic(parameterStruct, useModes, internalParams, postProInputs);


%% Linear transients:
% Calculate longitudinal stiffness
[~, ~, Kxk] = solver.calculateFx0(parameterStruct, postProInputs, internalParams, useModes, starVar, primeVar, incrVar);

% Calculate cornering stiffness
[~, ~, Kya, ~, ~, ~, ~, ~, ~] = solver.calculateFy0(parameterStruct, postProInputs, internalParams, useModes, starVar, primeVar, incrVar);

% Pack varinf
varinf.Kxk = Kxk;
varinf.Kya = Kya;

% Calculate relaxation lengths and stiffness
[cx, cy, sigmax, sigmay] = solver.calculateRelax(parameterStruct, postProInputs, varinf);

% Export relaxation length only in linear transients mode
if userDynamics~=2
    sigmax = 0;
    sigmay = 0;
end

%% Non Linear transients:
% Calculate contact patch
[TV, b, ~] =  solver.calculateContactPatch(parameterStruct, postProInputs, incrVar.dpi);
a2 = TV*2;
b2 = b*2;

% Contact patch relaxation length (equals half of the contact length)
sigma_c = max(TV,0.02); % Eqn 9.29 pag 412 (0.02 is hard coded to avoid division between 0 at low vertical loads check Epsilon_Lim in Besselink PhD) Sigma_min = Table 8.4 Page 400 from the book

% Carcass stiffness
Ccx = (Kxk*cx)/(Kxk - cx*TV); %(Eqn 25 - Paper)
Ccy = (Kya*cy)/(Kya - cy*TV); %(Eqn 25 - Paper)

if Fz == 0
    Ccx = cx;
    Ccy = cy;
end

% Carcass damping
Kcx = parameterStruct.DAMP_RESIDUAL * Ccx; %(NO IDEA)
Kcy = parameterStruct.DAMP_RESIDUAL * Ccy; %(NO IDEA)

== matlab function mfeval_CPI_LIB/MFeval CPI library/MFeval CPI/Flip Tyre7 ==
  data: in input; flipSide parameter; out output
function out = flipsSide(in, flipSide)
%#codegen

if flipSide
    out = -in;
else
    out = in;
end

== matlab function mfeval_CPI_LIB/MFeval CPI library/MFeval CPI/Flip Tyre4 ==
  data: in input; flipSide parameter; out output
function out = flipsSide(in, flipSide)
%#codegen

if flipSide
    out = -in;
else
    out = in;
end

== matlab function mfeval_CPI_LIB/MFeval CPI library/MFeval CPI/Flip Tyre1 ==
  data: in input; flipSide parameter; out output
function out = flipsSide(in, flipSide)
%#codegen

if flipSide
    out = -in;
else
    out = in;
end

== matlab function mfeval_CPI_LIB/MFeval CPI library/MFeval CPI/Steady State Calculator (mfeval) ==
  data: muRoad input; Fz input; kappa input; alpha input; p input; Vx input; omega input; gamma input; phit input; Vsy input; parameterStruct parameter; Fx output; userUseMode parameter; Fy output; Mx output; My output; Mz output; rho output; t output; mux output; muy output; Rl output; userDynamics parameter
function [Fx, Fy, Mx, My, Mz, rho, t, mux, muy, Rl] = steadystate(muRoad, Fz, kappa, alpha, p, Vx, omega, gamma, phit, Vsy, parameterStruct, userUseMode, userDynamics)
%#codegen

% Update mux and muy with muRoad
parameterStruct.LMUX = parameterStruct.LMUX*muRoad(1);
parameterStruct.LMUY = parameterStruct.LMUY*muRoad(2);

% Pack inputs
inputs = [Fz, kappa, alpha, gamma, phit, Vx, p, omega, Vsy];
      
% Call mfeval
solver = mfeval.Solver;
out = solver.fullCPI(parameterStruct, inputs, userUseMode, userDynamics);

% Eliminate NaNs
out(isnan(out)) = 0;

% Export
Fx = out(1);
Fy = out(2);
My = out(5);
Mx = out(4);
Mz = out(6);
rho = out(7);
Rl = out(8);
t = out(9);
mux = out(10);
muy = out(11);

== matlab function mfeval_CPI_LIB/MFeval CPI library/MFeval CPI/Flip Tyre2 ==
  data: in input; flipSide parameter; out output
function out = flipsSide(in, flipSide)
%#codegen

if flipSide
    out = -in;
else
    out = in;
end

== matlab function mfeval_CPI_LIB/MFeval CPI library/MFeval CPI/Flip Tyre ==
  data: in input; flipSide parameter; out output
function out = flipsSide(in, flipSide)
%#codegen

if flipSide
    out = -in;
else
    out = in;
end

== matlab function mfeval_CPI_LIB/MFeval CPI library/MFeval CPI/Flip Tyre3 ==
  data: in input; flipSide parameter; out output
function out = flipsSide(in, flipSide)
%#codegen

if flipSide
    out = -in;
else
    out = in;
end
